simulink model "spitest2"  (Simulink 7.4)
settings: Solver=FixedStepDiscrete  SolverMode=SingleTasking  StartTime=0.0  StopTime=10.0  FixedStep=0.001  RelTol=1e-3
libraries: dsPICdrivers x5
settings Model: Creator=staff  LastModifiedBy=staff
settings OptimizationCC: OptimizeModelRefInitCode=on  LifeSpan=1
settings RTWCC: SystemTargetFile=pic32.tlc  MakeCommand=make_CreateMPLAB  TemplateMakefile=pic32_gcc.tmf  PostCodeGenCommand=dsPIC_Compile()  Description=Embedded Target for Microchip dsPIC (real-time)  ProcessScript=pic32_make_rtw_hook
settings CodeAppCC: IgnoreCustomStorageClasses=off
settings STFCustomTargetCC: IncludeMdlTerminateFcn=off  CombineOutputUpdateFcns=on  SuppressErrorStatus=on  ERTCustomFileBanners=on  SupportContinuousTime=off  SupportNonInlinedSFcns=off  SystemTargetFile=pic32.tlc
settings ERTTargetCC: MultiwordLength=2048  ParMdlRefBuildCompliant=off  CompOptLevelCompliant=off  IncludeMdlTerminateFcn=off  SuppressErrorStatus=on  ERTFirstTimeCompliant=off  ModelStepFunctionPrototypeControlCompliant=off  CPPClassGenCompliant=off  InlinedParameterPlacement=NonHierarchical  ERTSrcFileBannerTemplate=dsPIC_code_template.cgt  ERTHdrFileBannerTemplate=dsPIC_code_template.cgt  ERTDataSrcFileTemplate=dsPIC_code_template.cgt  ERTDataHdrFileTemplate=dsPIC_code_template.cgt  ERTCustomFileTemplate=dsPIC_main.tlc  ConvertIfToSwitch=off
settings CustomProperty: DataType=string  Value=C:\PROGRA~1\MATLAB\R2009b\bin\win32\gmake

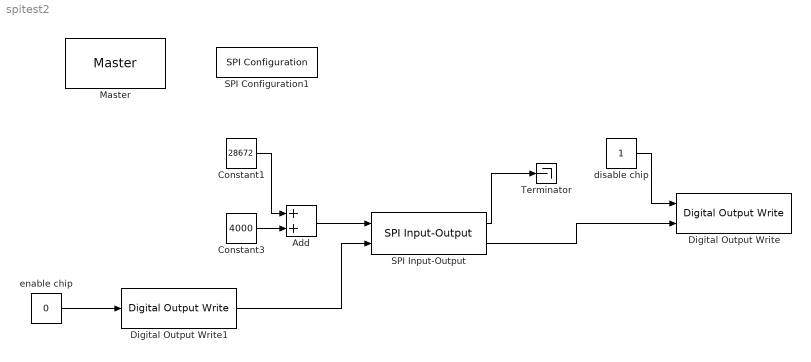
== system spitest2 ==
  Add : Sum  OutDataType=fixdt(1, 16)  OutScaling=2^-10
  Constant1 : Constant  Value=28672  OutDataTypeMode=uint16  OutDataType=fixdt(1, 16)  OutScaling=2^0  OutDataTypeStr=uint16
  Constant3 : Constant  Value=4000  OutDataTypeMode=uint16  OutDataType=fixdt(1, 16)  OutScaling=2^0  OutDataTypeStr=uint16
  Digital Output Write : dsPICdrivers/Digital I//O/Digital Output Write  Tag=dsPIC_Digital_Output  Priority=5  PORT=B  Pin=[2]  Simultaneous=off  OrderingInOutPopup=Input
  Digital Output Write1 : dsPICdrivers/Digital I//O/Digital Output Write  Tag=dsPIC_Digital_Output  Priority=5  PORT=B  Pin=[2]  Simultaneous=off  OrderingInOutPopup=Output
  Master : dsPICdrivers/Master  Tag=dsPIC_MASTER  Priority=1  TimeStepType=Timer1  picType=32MX360F512L  fcy=234375  Quartz_33f=8e6  PLLActive_33f=off  fcyDesired_33f=0  tmr1="[1  233  0.16]"  tmr1Info="Time Step : 0.0009984  ;   Error : 0.16%  PR1=233"  tmr2345="[0  0  0  0]"  tmr2345cfg=[-1 -1 -1 -1]  IOautoConf=on  typePort="[ 0   0   0   0   0   0   0   0   0   0   0   0   0   0   0   0   0   0  10   0   0   0   0   0   0   0   0   0   0   0   0   0   0   0   0   0   0   0   0   0   0   0   0   0   0   0   0   0   0   0   0   0   0   0   0   0   0   0   0   0   0   0   0   0   0   0   0   0   0   0   0   0   0   0   0   0   0   0   0   0   0   0   0   0   0   0  17  14  15   0   0   0   0   0   0   0   0   0   0   0   0   0   0   0   0   0   0   0   0   0   0   0 ]"  TRIS="[ 65535  65531  65535  65535  65535  65535  65535 ]"  ADPCFG=4  MasterBusyPort=None  MasterOverloadPort=None  FOSC=Quartz (XT - HS)  ClockSwitchMonitor=Both disabled  TempProtection_33f=TEMP_ON  FPBOR=<empty>  PWRT=disable  MCLR=<empty>  ICD=ICS_PGD1  JTAGEN=JTAGEN_OFF  PowerSave=off  OverrideFcy=off  NewFcy=1e6  PR2345="[65535  65535  65535  65535]"
  SPI Configuration1 : dsPICdrivers/SPI PORT/SPI Configuration  Tag=dsPIC_config_SPI  Priority=2  ConfigurationTime=At boot time (only once)  OrderingInOutPopup=None  SampleTime=-1  Frame_Enable=0  Frame_Sync=None  SPI=1  MODE=MASTER  USER_SCALER=1  StartEnable=Enable  SDO_EN=on  DATA_LENGTH=16 bits  SS_EN=off  SMP=End of bit  CKP=high  CKE=Active to Idle  Status="OK - Mode 0  -    Fsck= 234375Hz"
  SPI Input-Output : dsPICdrivers/SPI PORT/SPI Input-Output  Tag=dsPIC_SPI  SPI=1  INPUT=on  RESET_INPUT=off  OUTPUT=on  SPECIAL_SPI=Always Enable  DATA_LENGTH=16 bits  WAIT_INPUTDATA=on  OrderingInOutPopup=Input & Output  SampleTime=-1
  Terminator : Terminator
  disable chip : Constant  OutDataTypeMode=boolean  OutDataType=fixdt(1, 16)  OutScaling=2^0  OutDataTypeStr=boolean
  enable chip : Constant  Value=0  OutDataTypeMode=boolean  OutDataType=fixdt(1, 16)  OutScaling=2^0  OutDataTypeStr=boolean
  wires:
  Digital Output Write1/1 -> SPI Input-Output/2
  enable chip/1 -> Digital Output Write1/1
  disable chip/1 -> Digital Output Write/1
  SPI Input-Output/1 -> Terminator/1
  SPI Input-Output/2 -> Digital Output Write/2
  Constant1/1 -> Add/1
  Constant3/1 -> Add/2
  Add/1 -> SPI Input-Output/1
